simulink model "Inverter_pq_comp_sat_sim"  (R2023b)
settings: Solver=FixedStepDiscrete  StartTime=0.0  StopTime=2  RelTol=1e-3  EnableMultiTasking=on
InitFcn:
  | %% Definition of the parameters
  | 
  | Parameter_Definition
  | 
  | %% Damping
  | 
  | Rd = 3.9;
  | 
  | %% PRes Gains Calculation
  | 
  | % Definicao das grandezas
  | w_cl = 1j*2*pi*1200;  % Phase Crossing Frequency
  | no   = 1;           % Integral Resonant Constant
  | A    = 1;             % Carrier Amplitude
  | 
  | % Kp calculation
  | a0 = 1;
  | a1 = Rd*Cf;
  | b0 = 0;
  | b1 = Lf+Lg;
  | b2 = Rd*Lf*Cf+Rd*Lg*Cf;
  | b3 = Lf*Lg*Cf;
  | 
  | G_lcl = (a1*w_cl+a0)/(b3*w_cl^3+b2*w_cl^2+b1*w_cl+b0);
  | % G_lcl = 1/((Lf+Lg)*w_cl+Rf);
  | 
  | G_PWM = (1/A)*(1-w_cl*Ts/4)/(1+w_cl*Ts/4);
  | 
  | G_wc  = (Vdc/2)*(1/I_base)*G_lcl*G_PWM;
  | 
  | G_wc_abs = abs(G_wc);
  | 
  | Kp = 1/G_wc_abs;
  | 
  | % Discretized Controller Gains
  | ressonance_list = [1,5,7,11,13];
  | 
  | n_res = length(ressonance_list);
  | a = zeros(2,n_res);
  | b = zeros(2,n_res);
  | Ki_res = zeros(1,n_res);
  | 
  | % for i = 1:n_res
  | %   k = ressonance_list(i);
  | %   Ki_res(i) = (2.2*Kp)/(no*T_gr);
  | %   a(i) = (2*Ki_res(i)*Ts)/(4+((k*w_gr)^2)*Ts^2);
  | %   b(i) = (-8+2*((k*w_gr)^2)*Ts^2)/(4+((k*w_gr)^2)*Ts^2);
  | % end
  | 
  | % wc is the cutoff frequency/damping factor in rad/s
  | wc = 2;
  | 
  | for i = 1:n_res
  |   k = ressonance_list(i);
  |   wk = k * w_gr; % Resonant frequency for this harmonic
  | 
  |   Ki_res(i) = (2.2*Kp)/(0.8*no*T_gr);
  | 
  |   % 1. Calculate the common denominator
  |   den = 4 + 4*wc*Ts + (wk^2)*(Ts^2);
  | 
  |   % 2. Calculate the numerator terms (A coefficients for the input x)
  |   num_A0 = 2 * Ki_res(i) * wc * Ts;
  | 
  |   % 3. Calculate the denominator terms (B coefficients for the output y)
  |   num_B1 = -8 + 2*(wk^2)*(Ts^2);
  |   num_B2 = 4 - 4*wc*Ts + (wk^2)*(Ts^2);
  | 
  |   % 4. Normalize the coefficients
  |   a(1,i) = num_A0 / den;
  |   a(2,i) = -1*num_A0 / den;
  |   b(1,i) = num_B1 / den;
  |   b(2,i) = num_B2 / den;
  | end
values from neighbouring files (symbols this model uses):
  a1_sogi = single(2*(w0_sogi^2-c_sogi^2)/den0_sogi)    [Parameter_Definition.m]
  a2_sogi = single((c_sogi^2                 - k_sogi*w0_sogi*c_sogi                 + w0_sogi^2)/den0_sogi)    [Parameter_Definition.m]
  bD_sogi = single(k_sogi*w0_sogi*c_sogi/den0_sogi)    [Parameter_Definition.m]
  bQ_sogi = single(k_sogi*w0_sogi^2/den0_sogi)    [Parameter_Definition.m]
  Cdc = 1.5e-3    (= 0.0015)    [Parameter_Definition.m]
  Cf = 5e-6    (= 5e-06)    [Parameter_Definition.m]
  f_gr = 60    [Parameter_Definition.m]
  I_base = S_base/(sqrt(3)*V_gr)    [Parameter_Definition.m]
  Lf = 1e-3    (= 0.001)    [Parameter_Definition.m]
  Lg = 0.5e-3    (= 0.0005)    [Parameter_Definition.m]
  Rdc = 0.1/(2*pi*60*Cdc)    (= 0.176838825658)    [Parameter_Definition.m]
  Rf = 0.1*Xf    (= 0.0376991118431)    [Parameter_Definition.m]
  Rg = 0.1*Xg    (= 0.0188495559215)    [Parameter_Definition.m]
  S_base = S_rated    (= 1000)    [Parameter_Definition.m]
  Ts = 2*(4167)/100e6    (= 8.334e-05)    [Parameter_Definition.m]
  Tstep = Ts/1000    (= 8.334e-08)    [Parameter_Definition.m]
  V_base = sqrt(3)*V_gr    [Parameter_Definition.m]
  V_gr = 127    [Parameter_Definition.m]
  Vdc = 800    [Parameter_Definition.m]
  Vdc_base = Vdc    (= 800)    [Parameter_Definition.m]
  w_gr = 2*pi*f_gr    (= 376.991118431)    [Parameter_Definition.m]
undefined symbols (not defined in the file or in its folder): gH_LUT, gQ_LUT, gV_LUT, lH_vetor, lQ_vetor, lV_vetor
libraries: spsSeriesRLCBranchLib x22, spsIGBTDiodeLib x12, spsCurrentMeasurementLib x9, spsVoltageMeasurementLib x5, c2837xDlib x4, spsACVoltageSourceLib x3, spsGroundLib x3, spsDCVoltageSourceLib x2, spsTriangleGeneratorLib x1, simulink x1, eeRmsMeasurement x1, spsTHDLib x1
(part 1 of 3)
settings Model: SimulationMode=accelerator  ExtModeTrigDuration=8  Creator=AugustoMatheusdosSan  LastModifiedBy=engam
settings SolverCC: AutoInsertRateTranBlk=on
settings OptimizationCC: DefaultUnderspecifiedDataType=single  EnhancedBackFolding=on  PassReuseOutputArgsAs=Individual arguments  MaxStackSize=1024  OptimizeBlockOrder=speed  DifferentSizesBufferReuse=on  OptimizationCustomize=off  EfficientTunableParamExpr=on
settings DebuggingCC: ParameterPrecisionLossMsg=none  ParameterTunabilityLossMsg=error
settings HardwareCC: ProdBitPerChar=16  ProdBitPerInt=16  ProdBitPerPointer=32  ProdBitPerSizeT=32  ProdBitPerPtrDiffT=32  ProdLargestAtomicInteger=Integer  ProdLargestAtomicFloat=None  ProdWordSize=16  ProdLongLongMode=on  ProdHWDeviceType=Texas Instruments->C2000  HardwareBoardFeatureSet=SoCBlockset
settings ModelReferenceCC: ModelReferenceNumInstancesAllowed=Single
settings SFSimCC: MATLABDynamicMemAlloc=off
settings RTWCC: Description=Embedded Coder  SystemTargetFile=ert.tlc  HardwareBoard=TI Delfino F2837xD  TemplateMakefile=ert_default_tmf  Toolchain=Texas Instruments Code Composer Studio (C2000)  BuildConfiguration=Faster Runs  CodeProfilingSaveOptions=MetricsOnly
settings CodeAppCC: ForceParamTrailComments=on  IgnoreCustomStorageClasses=off  OperatorAnnotations=on  SimulinkDataObjDesc=on  SFDataObjDesc=on  InsertBlockDesc=on
settings ERTTargetCC: TargetLangStandard=C99 (ISO)  CodeReplacementLibrary=TI C28x  ExtModeTransport=4  ExtModeStaticAlloc=on  ExtModeAutomaticAllocSize=off  ExtModeStaticAllocSize=10000  ExtModeMexFile=ext_xcp  ExtModeIntrfLevel=Level2 - Open  EnableUserReplacementTypes=on

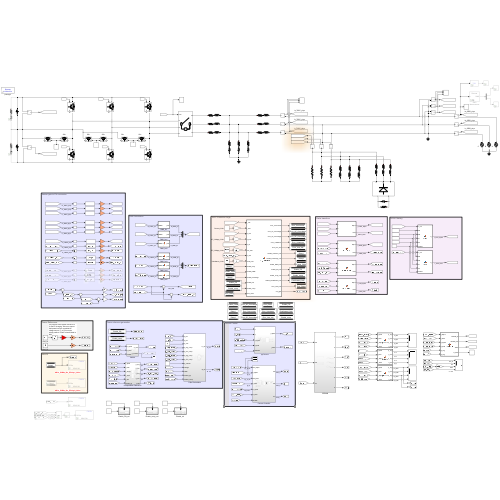
[thumbnail: Simulink's stored preview of the top-level diagram]
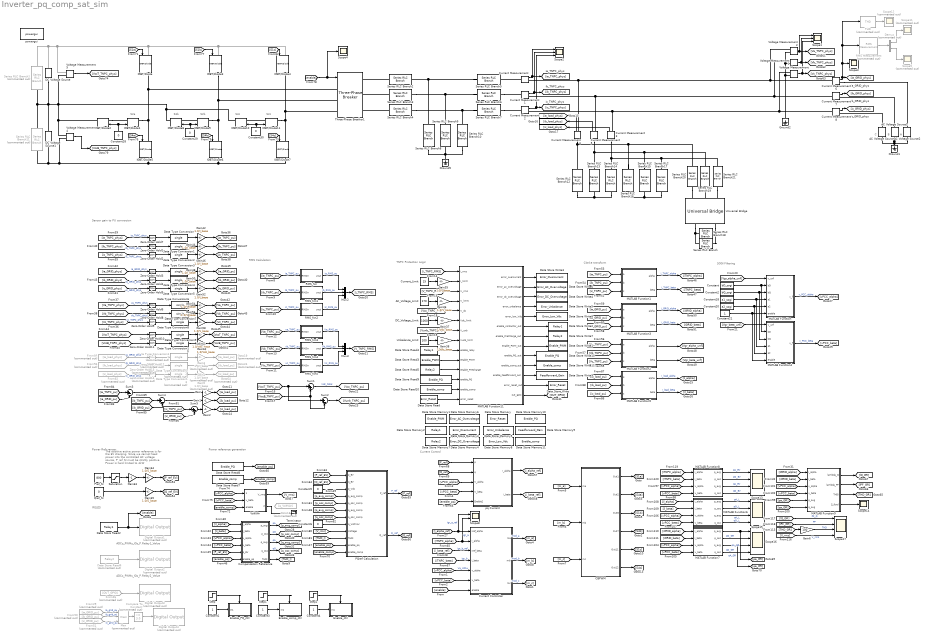
== system Inverter_pq_comp_sat_sim ==
  note: Power reference generation
  note: Current Control
  note: Power References
  note: The positive active power reference is for the EV charging. Since we cannot feed power into the controlled AC voltage source, P_ref_SI must be strictly positive. Power is hard limited to 4kW
  note: Sensor gain to PU conversion
  note: SOGI Filtering
  note: Clarke transform
  note: RELÉS
  note: ADCs_PWMs_IOs_P.Relay2_Value
  note: ADCs_PWMs_IOs_P.Relay1_Value
  note: RMS Calculation
  note: TNPC Protection Logic
  note: S3c
  note: S2b
  note: S2c
  note: S3b
  note: S2a
  note: C
  note: A
  note: B
  AC Voltage Source : spsACVoltageSourceLib/AC Voltage Source  Amplitude=V_gr*sqrt(2)  Phase=120  Frequency=f_gr  SampleTime=0  Measurements=None  BusType=swing  Pref=10e3  Qref=0  Qmin=-inf  Qmax=+inf
  AC Voltage Source1 : spsACVoltageSourceLib/AC Voltage Source  Amplitude=V_gr*sqrt(2)  Phase=-120  Frequency=f_gr  SampleTime=0  Measurements=None  BusType=swing  Pref=10e3  Qref=0  Qmin=-inf  Qmax=+inf
  AC Voltage Source2 : spsACVoltageSourceLib/AC Voltage Source  Amplitude=V_gr*sqrt(2)  Phase=0  Frequency=f_gr  SampleTime=0  Measurements=None  BusType=swing  Pref=10e3  Qref=0  Qmin=-inf  Qmax=+inf
  AC_Voltage_Limit : Constant  Value=170  OutDataTypeStr=single
  CBPWM : Subsystem
  Compare To Constant : simulink/Logic and Bit Operations/Compare To Constant  Commented=on  relop=<=  const=3.0  OutDataTypeStr=boolean
  Compensation Reference : Subsystem
  Constant : Constant  Value=bD_sogi
  Constant1 : Constant  OutDataTypeStr=single
  Constant18 : Constant  Value=a1_sogi
  Constant2 : Constant  Value=bQ_sogi
  Constant20 : Constant  Value=a2_sogi
  Constant21 : Constant
  Constant28 : Constant  Value=0
  Constant29 : Constant  Value=0
  Constant3 : Constant  OutDataTypeStr=single
  Constant30 : Constant  Value=0
  Constant4 : Constant  OutDataTypeStr=single
  Constant5 : Constant  Value=0  OutDataTypeStr=single
  Constant6 : Constant  Value=0  OutDataTypeStr=single
  Current Controller : Subsystem
  Current Measurement{,1..8} (9 alike) : spsCurrentMeasurementLib/Current Measurement  PhasorSimulation=off  OutputType=Complex  PSBequivalent=0
  Current_Limit : Constant  Value=15  OutDataTypeStr=single
  DC Voltage Source : spsDCVoltageSourceLib/DC Voltage Source  Amplitude=Vdc/2  Measurements=None
  DC Voltage Source1 : spsDCVoltageSourceLib/DC Voltage Source  Amplitude=Vdc/2  Measurements=None
  DC_Voltage_Limit : Constant  Value=1000  OutDataTypeStr=single
  Data Store Memory : DataStoreMemory  DataStoreName=Error_Reset  WriteAfterWriteMsg=warning  ShowAdditionalParam=off  OutDataTypeStr=single
  Data Store Memory1 : DataStoreMemory  DataStoreName=Enable_PWM  WriteAfterWriteMsg=warning  ShowAdditionalParam=off  OutDataTypeStr=single
  Data Store Memory10 : DataStoreMemory  DataStoreName=Enable_PQ  WriteAfterWriteMsg=warning  ShowAdditionalParam=off  OutDataTypeStr=single
  Data Store Memory11 : DataStoreMemory  DataStoreName=Enable_comp  WriteAfterWriteMsg=warning  ShowAdditionalParam=off  OutDataTypeStr=single
  Data Store Memory2 : DataStoreMemory  DataStoreName=Relay1  WriteAfterWriteMsg=warning  ShowAdditionalParam=off  OutDataTypeStr=single
  Data Store Memory3 : DataStoreMemory  DataStoreName=Error_Overcurrent  WriteAfterWriteMsg=warning  ShowAdditionalParam=off  OutDataTypeStr=single
  Data Store Memory4 : DataStoreMemory  DataStoreName=Error_DC_Overvoltage  WriteAfterWriteMsg=warning  ShowAdditionalParam=off  OutDataTypeStr=single
  Data Store Memory5 : DataStoreMemory  DataStoreName=Error_Unbalance  WriteAfterWriteMsg=warning  ShowAdditionalParam=off  OutDataTypeStr=single
  Data Store Memory6 : DataStoreMemory  DataStoreName=Error_AC_Overvoltage  WriteAfterWriteMsg=warning  ShowAdditionalParam=off  OutDataTypeStr=single
  Data Store Memory7 : DataStoreMemory  DataStoreName=Relay2  WriteAfterWriteMsg=warning  ShowAdditionalParam=off  OutDataTypeStr=single
  Data Store Memory8 : DataStoreMemory  DataStoreName=Error_Low_Vdc  WriteAfterWriteMsg=warning  ShowAdditionalParam=off  OutDataTypeStr=single
  Data Store Memory9 : DataStoreMemory  DataStoreName=Feedforward_Gain  WriteAfterWriteMsg=warning  ShowAdditionalParam=off  OutDataTypeStr=single
  Data Store Read : DataStoreRead  DataStoreName=Error_Reset  SampleTime=Ts  IndexOptions=Index vector (dialog)  Indices=1  OutputSizes=1
  Data Store Read10 : DataStoreRead  DataStoreName=Enable_comp  SampleTime=Ts  IndexOptions=Index vector (dialog)  Indices=1  OutputSizes=1
  Data Store Read2 : DataStoreRead  DataStoreName=Relay1  SampleTime=Ts  IndexOptions=Index vector (dialog)  Indices=1  OutputSizes=1
  Data Store Read3 : DataStoreRead  DataStoreName=Enable_PWM  SampleTime=Ts  IndexOptions=Index vector (dialog)  Indices=1  OutputSizes=1
  Data Store Read4 : DataStoreRead  DataStoreName=Relay1  SampleTime=Ts  IndexOptions=Index vector (dialog)  Indices=1  OutputSizes=1
  Data Store Read5 : DataStoreRead  DataStoreName=Relay2  SampleTime=Ts  IndexOptions=Index vector (dialog)  Indices=1  OutputSizes=1
  Data Store Read6 : DataStoreRead  Commented=on  DataStoreName=Relay2  IndexOptions=Index vector (dialog)  Indices=1  OutputSizes=1
  Data Store Read7 : DataStoreRead  DataStoreName=Enable_comp  SampleTime=Ts  IndexOptions=Index vector (dialog)  Indices=1  OutputSizes=1
  Data Store Read8 : DataStoreRead  DataStoreName=Enable_PQ  SampleTime=Ts  IndexOptions=Index vector (dialog)  Indices=1  OutputSizes=1
  Data Store Read9 : DataStoreRead  DataStoreName=Enable_PQ  SampleTime=Ts  IndexOptions=Index vector (dialog)  Indices=1  OutputSizes=1
  Data Store Write : DataStoreWrite  DataStoreName=Error_Reset  SampleTime=Ts  IndexOptions=Index vector (dialog)  Indices=1  OutputSizes=1
  Data Store Write1 : DataStoreWrite  DataStoreName=Enable_PWM  SampleTime=Ts  IndexOptions=Index vector (dialog)  Indices=1  OutputSizes=1
  Data Store Write10 : DataStoreWrite  DataStoreName=Enable_PQ  SampleTime=Ts  IndexOptions=Index vector (dialog)  Indices=1  OutputSizes=1
  Data Store Write11 : DataStoreWrite  DataStoreName=Enable_comp  SampleTime=Ts  IndexOptions=Index vector (dialog)  Indices=1  OutputSizes=1
  Data Store Write2 : DataStoreWrite  DataStoreName=Relay1  SampleTime=Ts  IndexOptions=Index vector (dialog)  Indices=1  OutputSizes=1
  Data Store Write3 : DataStoreWrite  DataStoreName=Error_Overcurrent  SampleTime=Ts  IndexOptions=Index vector (dialog)  Indices=1  OutputSizes=1
  Data Store Write4 : DataStoreWrite  DataStoreName=Error_DC_Overvoltage  SampleTime=Ts  IndexOptions=Index vector (dialog)  Indices=1  OutputSizes=1
  Data Store Write5 : DataStoreWrite  DataStoreName=Error_Unbalance  SampleTime=Ts  IndexOptions=Index vector (dialog)  Indices=1  OutputSizes=1
  Data Store Write6 : DataStoreWrite  DataStoreName=Error_AC_Overvoltage  SampleTime=Ts  IndexOptions=Index vector (dialog)  Indices=1  OutputSizes=1
  Data Store Write7 : DataStoreWrite  DataStoreName=Relay2  SampleTime=Ts  IndexOptions=Index vector (dialog)  Indices=1  OutputSizes=1
  Data Store Write8 : DataStoreWrite  DataStoreName=Error_Low_Vdc  SampleTime=Ts  IndexOptions=Index vector (dialog)  Indices=1  OutputSizes=1
  Data Store Write9 : DataStoreWrite  DataStoreName=Feedforward_Gain  SampleTime=Ts  IndexOptions=Index vector (dialog)  Indices=1  OutputSizes=1
  Data Type Conversion{,1..10} (11 alike) : DataTypeConversion  OutDataTypeStr=single  SaturateOnIntegerOverflow=off  RndMeth=Floor
  Data Type Conversion11 : DataTypeConversion  Commented=on  OutDataTypeStr=single  SaturateOnIntegerOverflow=off  RndMeth=Floor
  Data Type Conversion12 : DataTypeConversion  Commented=on  OutDataTypeStr=single  SaturateOnIntegerOverflow=off  RndMeth=Floor
  Data Type Conversion13 : DataTypeConversion  Commented=on  OutDataTypeStr=single  SaturateOnIntegerOverflow=off  RndMeth=Floor
  Demux : Demux  Commented=on  Outputs=2
  Digital Output1 : c2837xDlib/Digital Output  Commented=on  GPIO_Number=GPIO32~GPIO39  GPIO_Bit0=off  GPIO_BIT0_Toggle=off  GPIO_Bit1=off  GPIO_BIT1_Toggle=off  GPIO_Bit2=off  GPIO_BIT2_Toggle=off  GPIO_Bit3=on  GPIO_BIT3_Toggle=off  GPIO_Bit4=off  GPIO_BIT4_Toggle=off  GPIO_Bit5=off  GPIO_BIT5_Toggle=off  GPIO_Bit6=off  GPIO_BIT6_Toggle=off  GPIO_Bit7=off  GPIO_BIT7_Toggle=off
  Digital Output2 : c2837xDlib/Digital Output  Commented=on  GPIO_Number=GPIO32~GPIO39  GPIO_Bit0=off  GPIO_BIT0_Toggle=off  GPIO_Bit1=off  GPIO_BIT1_Toggle=off  GPIO_Bit2=off  GPIO_BIT2_Toggle=off  GPIO_Bit3=off  GPIO_BIT3_Toggle=off  GPIO_Bit4=off  GPIO_BIT4_Toggle=off  GPIO_Bit5=on  GPIO_BIT5_Toggle=off  GPIO_Bit6=off  GPIO_BIT6_Toggle=off  GPIO_Bit7=off  GPIO_BIT7_Toggle=off
  Digital Output3 : c2837xDlib/Digital Output  Commented=on  GPIO_Number=GPIO64~GPIO71  GPIO_Bit0=off  GPIO_BIT0_Toggle=off  GPIO_Bit1=off  GPIO_BIT1_Toggle=off  GPIO_Bit2=off  GPIO_BIT2_Toggle=off  GPIO_Bit3=on  GPIO_BIT3_Toggle=off  GPIO_Bit4=off  GPIO_BIT4_Toggle=off  GPIO_Bit5=off  GPIO_BIT5_Toggle=off  GPIO_Bit6=off  GPIO_BIT6_Toggle=off  GPIO_Bit7=off  GPIO_BIT7_Toggle=off
  Digital Output4 : c2837xDlib/Digital Output  Commented=on  GPIO_Number=GPIO64~GPIO71  GPIO_Bit0=off  GPIO_BIT0_Toggle=off  GPIO_Bit1=off  GPIO_BIT1_Toggle=off  GPIO_Bit2=off  GPIO_BIT2_Toggle=off  GPIO_Bit3=off  GPIO_BIT3_Toggle=off  GPIO_Bit4=on  GPIO_BIT4_Toggle=off  GPIO_Bit5=off  GPIO_BIT5_Toggle=off  GPIO_Bit6=off  GPIO_BIT6_Toggle=off  GPIO_Bit7=off  GPIO_BIT7_Toggle=off
  Enable_PQ_ctrl : Subsystem  TreatAsAtomicUnit=on
  Enable_comp_ctrl : Subsystem  TreatAsAtomicUnit=on
  Enable_ctrl : Subsystem  TreatAsAtomicUnit=on
  From26 : From  Commented=on  GotoTag=OUT_GPIO
  From29 : From  Commented=on  GotoTag=ia_GRID_pu
  From50 : From  Commented=on  GotoTag=ib_GRID_pu
  From51 : From  Commented=on  GotoTag=ic_GRID_pu
  From92 : From  Commented=on  GotoTag=ic_load_phys
  From93 : From  Commented=on  GotoTag=ia_load_phys
  From94 : From  Commented=on  GotoTag=ib_load_phys
  Gain{,1..2,63} (4 alike) : Gain  Gain=-1
  Gain3 : Gain  Commented=on  Gain=1.0/I_base
  Gain{35,42,44,46,48,50,52} (7 alike) : Gain  Gain=1.0/I_base
  Gain{36,54,56,58} (4 alike) : Gain  Gain=1.0/V_base
  Gain37 : Gain  Gain=1/Vdc_base
  Gain38 : Gain  Gain=1/Vdc_base
  Gain4 : Gain  Commented=on  Gain=1.0/I_base
  Gain5 : Gain  Commented=on  Gain=1.0/I_base
  Gain6 : Gain  Gain=100
  Gain61 : Gain  Gain=1.0/Vdc_base
  Gain62 : Gain  Gain=1.0/Vdc_base
  Gain64 : Gain  Gain=1.0/S_base
  Gain65 : Gain  Gain=1.0/S_base
  Goto18 : Goto  Commented=on  GotoTag=q_VoltVAr
  Goto19 : Goto  Commented=on  GotoTag=ia_load_pu
  Goto24 : Goto  Commented=on  GotoTag=ib_load_pu
  Goto64 : Goto  Commented=on  GotoTag=ic_load_pu
  Ground1 : spsGroundLib/Ground  LConnTagsString=a
  Ground2 : spsGroundLib/Ground  LConnTagsString=a
  Ground5 : spsGroundLib/Ground  LConnTagsString=a
  IGBT/Diode{,1..11} (12 alike) : spsIGBTDiodeLib/IGBT//Diode  Ron=Rfet  Rs=1e5  Cs=inf  Measurements=on
  MATLAB Function : MATLAB Function  TreatAsAtomicUnit=on
  MATLAB Function1 : MATLAB Function  TreatAsAtomicUnit=on
  MATLAB Function11 : MATLAB Function  TreatAsAtomicUnit=on
  MATLAB Function2 : MATLAB Function  TreatAsAtomicUnit=on
  MATLAB Function3 : MATLAB Function  TreatAsAtomicUnit=on
  MATLAB Function4 : MATLAB Function  TreatAsAtomicUnit=on
  MATLAB Function5 : MATLAB Function  TreatAsAtomicUnit=on
  MATLAB Function6 : MATLAB Function  TreatAsAtomicUnit=on
  MATLAB Function7 : MATLAB Function  TreatAsAtomicUnit=on
  MATLAB Function8 : MATLAB Function  TreatAsAtomicUnit=on
  MATLAB Function9 : MATLAB Function  TreatAsAtomicUnit=on
  Max : MinMax  Commented=on  Function=max  Inputs=3
  Mux2 : Mux  Inputs=3
  Mux3 : Mux  Inputs=3
  PQref Calculation : Subsystem
  Pref_SI : Constant  Value=800  OutDataTypeStr=single
  Qref_SI : Constant  Value=0  OutDataTypeStr=single
  RMS Measurement : eeRmsMeasurement/RMS Measurement  Commented=on  LabelModeActiveChoice=Harmonic  F=60  SpecifyHarmonics=on  K=[1:40]  Ts=Ts
      settings: LibrarySourceBlock=|
      | ee_sl_lib/Measurements/RMS
      | Measurement
  RMS_fcn : MATLAB Function  TreatAsAtomicUnit=on
  RMS_fcn1 : MATLAB Function  TreatAsAtomicUnit=on
  RMS_fcn2 : MATLAB Function  TreatAsAtomicUnit=on
  RMS_fcn3 : MATLAB Function  TreatAsAtomicUnit=on
  RMS_fcn4 : MATLAB Function  TreatAsAtomicUnit=on
  RMS_fcn5 : MATLAB Function  TreatAsAtomicUnit=on
  Saturation : Saturate  UpperLimit=4000  LowerLimit=0
  Scope1 : Scope  NumInputPorts=3
  Scope11 : Scope  Commented=on
  Scope12 : Scope  Commented=on
  Scope{13,15..17} (4 alike) : Scope  NumInputPorts=4
  Scope14 : Scope
  Scope2 : Scope  NumInputPorts=3
  Scope3 : Scope
  Scope4 : Scope
  Scope5 : Scope  Commented=on
  Scope8 : Scope  NumInputPorts=2
  Series RLC Branch : spsSeriesRLCBranchLib/Series RLC Branch  LConnTagsString=__new0  RConnTagsString=__new0  BranchType=R  Resistance=400  Inductance=1e-3  SetiL0=off  InitialCurrent=0  Capacitance=1e-6  Setx0=off  InitialVoltage=0  Measurements=None
  Series RLC Branch1 : spsSeriesRLCBranchLib/Series RLC Branch  Commented=on  LConnTagsString=__new0  RConnTagsString=__new0  BranchType=RC  Resistance=Rdc*0.1  Inductance=Cdc  SetiL0=off  InitialCurrent=0  Capacitance=Cdc  Setx0=on  InitialVoltage=Vdc/2  Measurements=None
  Series RLC Branch10 : spsSeriesRLCBranchLib/Series RLC Branch  LConnTagsString=__new0  RConnTagsString=__new0  BranchType=RC  Resistance=Rd  Inductance=5e-3  SetiL0=off  InitialCurrent=0  Capacitance=Cf  Setx0=off  InitialVoltage=0  Measurements=None
  Series RLC Branch11 : spsSeriesRLCBranchLib/Series RLC Branch  Commented=on  LConnTagsString=__new0  RConnTagsString=__new0  BranchType=RC  Resistance=Rdc*0.1  Inductance=Cdc  SetiL0=off  InitialCurrent=0  Capacitance=Cdc  Setx0=on  InitialVoltage=Vdc/2  Measurements=None
  Series RLC Branch12 : spsSeriesRLCBranchLib/Series RLC Branch  LConnTagsString=__new0  RConnTagsString=__new0  BranchType=R  Resistance=80*160/240  Inductance=5e-3  SetiL0=off  InitialCurrent=0  Capacitance=inf  Setx0=off  InitialVoltage=0  Measurements=None
  Series RLC Branch13 : spsSeriesRLCBranchLib/Series RLC Branch  LConnTagsString=__new0  RConnTagsString=__new0  BranchType=R  Resistance=80*160/240  Inductance=5e-3  SetiL0=off  InitialCurrent=0  Capacitance=inf  Setx0=off  InitialVoltage=0  Measurements=None
  Series RLC Branch14 : spsSeriesRLCBranchLib/Series RLC Branch  LConnTagsString=__new0  RConnTagsString=__new0  BranchType=R  Resistance=80*160/240  Inductance=5e-3  SetiL0=off  InitialCurrent=0  Capacitance=inf  Setx0=off  InitialVoltage=0  Measurements=None
  Series RLC Branch15 : spsSeriesRLCBranchLib/Series RLC Branch  LConnTagsString=__new0  RConnTagsString=__new0  BranchType=RL  Resistance=5.47  Inductance=188.7e-3  SetiL0=off  InitialCurrent=0  Capacitance=inf  Setx0=off  InitialVoltage=0  Measurements=None
  Series RLC Branch16 : spsSeriesRLCBranchLib/Series RLC Branch  LConnTagsString=__new0  RConnTagsString=__new0  BranchType=RL  Resistance=5.47  Inductance=188.7e-3  SetiL0=off  InitialCurrent=0  Capacitance=inf  Setx0=off  InitialVoltage=0  Measurements=None
  Series RLC Branch17 : spsSeriesRLCBranchLib/Series RLC Branch  LConnTagsString=__new0  RConnTagsString=__new0  BranchType=RL  Resistance=5.47  Inductance=188.7e-3  SetiL0=off  InitialCurrent=0  Capacitance=inf  Setx0=off  InitialVoltage=0  Measurements=None
  Series RLC Branch18 : spsSeriesRLCBranchLib/Series RLC Branch  LConnTagsString=__new0  RConnTagsString=__new0  BranchType=C  Resistance=(54/pi^2)*(127^2/1e3)  Inductance=1e-3  SetiL0=off  InitialCurrent=0  Capacitance=5e-3  Setx0=off  InitialVoltage=0  Measurements=None
  Series RLC Branch19 : spsSeriesRLCBranchLib/Series RLC Branch  LConnTagsString=__new0  RConnTagsString=__new0  BranchType=RL  Resistance=0.1*2*pi*60*1e-3  Inductance=1e-3  SetiL0=off  InitialCurrent=0  Capacitance=5e-6  Setx0=off  InitialVoltage=0  Measurements=None
  Series RLC Branch2 : spsSeriesRLCBranchLib/Series RLC Branch  LConnTagsString=__new0  RConnTagsString=__new0  BranchType=RL  Resistance=Rf  Inductance=Lf  SetiL0=off  InitialCurrent=0  Capacitance=1e-6  Setx0=off  InitialVoltage=0  Measurements=None
  Series RLC Branch20 : spsSeriesRLCBranchLib/Series RLC Branch  LConnTagsString=__new0  RConnTagsString=__new0  BranchType=RL  Resistance=0.1*2*pi*60*1e-3  Inductance=1e-3  SetiL0=off  InitialCurrent=0  Capacitance=5e-6  Setx0=off  InitialVoltage=0  Measurements=None
  Series RLC Branch21 : spsSeriesRLCBranchLib/Series RLC Branch  LConnTagsString=__new0  RConnTagsString=__new0  BranchType=RL  Resistance=0.1*2*pi*60*1e-3  Inductance=1e-3  SetiL0=off  InitialCurrent=0  Capacitance=5e-6  Setx0=off  InitialVoltage=0  Measurements=None
  Series RLC Branch3 : spsSeriesRLCBranchLib/Series RLC Branch  LConnTagsString=__new0  RConnTagsString=__new0  BranchType=RL  Resistance=Rf  Inductance=Lf  SetiL0=off  InitialCurrent=0  Capacitance=1e-6  Setx0=off  InitialVoltage=0  Measurements=None
  Series RLC Branch4 : spsSeriesRLCBranchLib/Series RLC Branch  LConnTagsString=__new0  RConnTagsString=__new0  BranchType=RL  Resistance=Rf  Inductance=Lf  SetiL0=off  InitialCurrent=0  Capacitance=1e-6  Setx0=off  InitialVoltage=0  Measurements=None
  Series RLC Branch5 : spsSeriesRLCBranchLib/Series RLC Branch  LConnTagsString=__new0  RConnTagsString=__new0  BranchType=RL  Resistance=Rg  Inductance=Lg  SetiL0=off  InitialCurrent=0  Capacitance=1e-6  Setx0=off  InitialVoltage=0  Measurements=None
  Series RLC Branch6 : spsSeriesRLCBranchLib/Series RLC Branch  LConnTagsString=__new0  RConnTagsString=__new0  BranchType=RL  Resistance=Rg  Inductance=Lg  SetiL0=off  InitialCurrent=0  Capacitance=1e-6  Setx0=off  InitialVoltage=0  Measurements=None
  Series RLC Branch7 : spsSeriesRLCBranchLib/Series RLC Branch  LConnTagsString=__new0  RConnTagsString=__new0  BranchType=RL  Resistance=Rg  Inductance=Lg  SetiL0=off  InitialCurrent=0  Capacitance=1e-6  Setx0=off  InitialVoltage=0  Measurements=None
  Series RLC Branch8 : spsSeriesRLCBranchLib/Series RLC Branch  LConnTagsString=__new0  RConnTagsString=__new0  BranchType=RC  Resistance=Rd  Inductance=5e-3  SetiL0=off  InitialCurrent=0  Capacitance=Cf  Setx0=off  InitialVoltage=0  Measurements=None
  Series RLC Branch9 : spsSeriesRLCBranchLib/Series RLC Branch  LConnTagsString=__new0  RConnTagsString=__new0  BranchType=RC  Resistance=Rd  Inductance=5e-3  SetiL0=off  InitialCurrent=0  Capacitance=Cf  Setx0=off  InitialVoltage=0  Measurements=None
  Step : Step  OutDataTypeStr=single  SampleTime=Ts
  Step1 : Step  Time=1.5  OutDataTypeStr=single  SampleTime=Ts
  Step2 : Step  Time=0.5  OutDataTypeStr=single  SampleTime=Ts
  Sum1 : Sum  Inputs=|++
  Sum{2..5} (4 alike) : Sum  Inputs=|+-
  THD : spsTHDLib/THD  Commented=on  Freq=60  Ts=Tstep
  Terminator : Terminator
  Three-Phase Breaker1 : spsThreePhaseBreakerLib/Three-Phase Breaker  InitialState=open  SwitchA=on  SwitchB=on  SwitchC=on  SwitchTimes="[1/60  5/60]"  External=on  BreakerResistance=0.001  SnubberResistance=1e6  SnubberCapacitance=inf  Measurements=None
  Unbalance_Limit : Constant  Value=100  OutDataTypeStr=single
  Universal Bridge : spsUniversalBridgeLib/Universal Bridge  Arms=3  SnubberResistance=1e5  SnubberCapacitance=inf  Device=Diodes  Ron=1e-3  Lon=0  ForwardVoltages="[  0  0  ]"  ForwardVoltage=0  GTOparameters=[ 10e-6 , 20e-6 ]  IGBTparameters=[ 1e-6 , 2e-6 ]  Measurements=None  Measurements_2=None  converterType=Rectifier
  VoltVAr : Subsystem
  Voltage Measurement{,1..2,4..5} (5 alike) : spsVoltageMeasurementLib/Voltage Measurement  PhasorSimulation=off  OutputType=Complex  PSBequivalent=0
  Zero-Order Hold{1..11} (11 alike) : ZeroOrderHold  SampleTime=Ts
  Zero-Order Hold12 : ZeroOrderHold  Commented=on  SampleTime=Ts
  Zero-Order Hold13 : ZeroOrderHold  Commented=on  SampleTime=Ts
  Zero-Order Hold14 : ZeroOrderHold  Commented=on  SampleTime=Ts
  powergui : sps_lib/powergui  Priority=1  SimulationMode=Discrete  SampleTime=Tstep  frequency=60  Iterations=50  frequencyindice=60  Pbase=100e6  ErrMax=1e-4  UnitsV=kV  UnitsW=MW  buscounter=0  FunctionMessages=off  echomessages=off  EnableUseOfTLC=off  CurrentSourceSwitches=off  DisableSnubberDevices=off  DisableRonSwitches=off  DisableVfSwitches=off  DisplayEquations=off  AutomaticDiscreteSolvers=off  SolverType=Tustin/Backward Euler (TBE)  Interpol=off  ExternalGateDelay=off  methode=off  Ts=100  x0status=blocks  SPID=on  SwTol=0  HookPort=off  NonlinearTolerance=1e-4  nMaxIteration=100  ContinueOnMaxIteration=off  RestoreLinks=warning  ResistiveCurrentMeasurement=off  Frange=[0:2:500]  Ylog=off  Xlog=on  ShowGrid=off  save=off  variable=ZData  structure=0  ZoomFFT=off  StartTime=0.0  cycles=1  DisplayStyle=1  fundamental=60  FreqAxis=off  MaxFrequency=1000  frequencyindicesteady=1  RmsSteady=1  display=off
  pq Current : Subsystem
  wires:
  [iTNPC_alpha] -> Scope8/2, Current Controller/2(i_alpha)  "igr_a"
  [i_alpha_ref] -> Scope8/1, Current Controller/1(iref_alpha)  "igr_a_ref"
  [iTNPC_beta] -> Current Controller/4(i_beta)  "igr_b"
  [i_beta_ref] -> Current Controller/3(iref_beta)  "igr_b_ref"
  Current Controller/3(mc) -> [m_c]  "mod_c"
  Data Store Read6/1 -> Digital Output2/1
  Current Controller/2(mb) -> [m_b]  "mod_b"
  [enable] -> Current Controller/7(enable)
  Current Controller/1(ma) -> [m_a]  "mod_a"
  Data Store Read/1 -> MATLAB Function11/14(error_reset)
  [ib_TNPC_pu] -> RMS_fcn1/1(RMSin)  "ib_TNPC_pu"
  Data Store Read5/1 -> MATLAB Function11/11(enable_PreCharge)
  AC_Voltage_Limit/1 -> Gain36/1
  [ia_TNPC_pu] -> RMS_fcn/1(RMSin)  "ia_TNPC_pu"
  [VccB_TNPC_pu] -> Sum1/2, Sum2/2
  Data Store Read3/1 -> MATLAB Function11/10(enable_PWM)
  DC_Voltage_Limit/1 -> Gain37/1
  Gain35/1 -> MATLAB Function11/2(I_limit)
  Mux2/1 -> [i_TNPC_RMS]
  Unbalance_Limit/1 -> Gain38/1
  MATLAB Function11/8(enable_PWM_out) -> Data Store Write1/1
  [ic_TNPC_pu] -> RMS_fcn2/1(RMSin)  "ic_TNPC_pu"
  [Vcc_TNPC_pu] -> MATLAB Function11/5(V_dc)
  Gain36/1 -> MATLAB Function11/4(V_limit)
  MATLAB Function11/1(error_overcurrent) -> Data Store Write3/1
  [V_TNPC_RMS] -> MATLAB Function11/3(V_rms)
  Sum2/1 -> [Vunb_TNPC_pu]
  Gain38/1 -> MATLAB Function11/8(Vunb_limit)
  Gain37/1 -> MATLAB Function11/6(Vdc_limit)
  Data Store Read4/1 -> MATLAB Function11/9(enable_relay)
  Current_Limit/1 -> Gain35/1
  MATLAB Function11/7(enable_PreCharge_out) -> Data Store Write7/1
  MATLAB Function11/6(enable_contactor_out) -> Data Store Write2/1
  [i_TNPC_RMS] -> MATLAB Function11/1(i_rms)
  Sum1/1 -> [Vcc_TNPC_pu]  "Vdc_total"
  [Vunb_TNPC_pu] -> MATLAB Function11/7(V_unb)
  [VccT_TNPC_pu] -> Sum1/1, Sum2/1
  MATLAB Function11/12(error_reset_out) -> Data Store Write/1
  MATLAB Function11/3(error_dc_overvoltage) -> Data Store Write4/1
  MATLAB Function11/4(error_unbalance) -> Data Store Write5/1
  RMS_fcn/1(yout) -> Mux2/1  "ia_RMS_pu"
  RMS_fcn1/1(yout) -> Mux2/2  "ib_RMS_pu"
  RMS_fcn2/1(yout) -> Mux2/3  "ic_RMS_pu"
  [Va_TNPC_pu] -> RMS_fcn3/1(RMSin)  "va_TNPC_pu"
  [Vc_TNPC_pu] -> RMS_fcn5/1(RMSin)  "vc_TNPC_pu"
  [Vb_TNPC_pu] -> RMS_fcn4/1(RMSin)  "vb_TNPC_pu"
  RMS_fcn4/1(yout) -> Mux3/2  "Vb_RMS_pu"
  RMS_fcn3/1(yout) -> Mux3/1  "Va_RMS_pu"
  RMS_fcn5/1(yout) -> Mux3/3  "Vc_RMS_pu"
  Mux3/1 -> [V_TNPC_RMS]
  MATLAB Function11/2(error_ac_overvoltage) -> Data Store Write6/1
  MATLAB Function11/5(error_low_Vdc) -> Data Store Write8/1
  MATLAB Function11/13(out_gpio) -> [OUT_GPIO]
  From26/1 -> Digital Output3/1
  [vPCC_alpha] -> Current Controller/5(v_alpha)  "Va_inPLL"
  [vPCC_beta] -> Current Controller/6(v_beta)
  Data Store Read2/1 -> [enable], Digital Output1/1
  Compare To Constant/1 -> Digital Output4/1
  MATLAB Function11/11(enable_Feedforward_out) -> Data Store Write9/1
  From29/1 -> Max/1  "ia_grid_pu"
  Max/1 -> Compare To Constant/1
  From50/1 -> Max/2  "ib_grid_pu"
  From51/1 -> Max/3  "ic_grid_pu"
  [ia_TNPC_pu] -> MATLAB Function1/1(a)
  [ib_TNPC_pu] -> MATLAB Function1/2(b)
  [ic_TNPC_pu] -> MATLAB Function1/3(c)
  [Va_TNPC_pu] -> MATLAB Function2/1(a)
  [Vb_TNPC_pu] -> MATLAB Function2/2(b)
  [Vc_TNPC_pu] -> MATLAB Function2/3(c)
  MATLAB Function1/2(beta) -> [iTNPC_beta]  "i_TNPC_beta"
  MATLAB Function1/1(alpha) -> [iTNPC_alpha]  "i_TNPC_alpha"
  MATLAB Function2/1(alpha) -> [Vgr_alpha_unf]
  MATLAB Function2/2(beta) -> [Vgr_beta_unf]
  [ib_GRID_pu] -> MATLAB Function3/2(b)
  [ia_GRID_pu] -> MATLAB Function3/1(a)
  MATLAB Function3/2(beta) -> [iGRID_beta]  "i_GRID_beta"
  MATLAB Function3/1(alpha) -> [iGRID_alpha]  "i_GRID_alpha"
  [ic_GRID_pu] -> MATLAB Function3/3(c)
  [Vgr_beta_unf] -> MATLAB Function4/1(v_unf)
  [Vgr_alpha_unf] -> MATLAB Function/1(v_unf)
  MATLAB Function4/1(v_f) -> [vPCC_beta]  "v_PCC_beta"
  MATLAB Function/1(v_f) -> [vPCC_alpha]  "v_PCC_alpha"
  Constant/1 -> MATLAB Function4/2(bD), MATLAB Function/2(bD)
  Constant2/1 -> MATLAB Function4/3(bQ), MATLAB Function/3(bQ)
  Constant18/1 -> MATLAB Function4/4(a1), MATLAB Function/4(a1)
  Constant20/1 -> MATLAB Function4/5(a2), MATLAB Function/5(a2)
  Constant21/1 -> MATLAB Function4/6(enable), MATLAB Function/6(enable)
  [enable_pq] -> Compensation Reference/6(enable_pq)
  Compensation Reference/3(q_avg) -> [q_avg_comp]  "qA"
  [vPCC_beta] -> Compensation Reference/4(v_beta)
  Compensation Reference/4(q_osc) -> [q_osc_comp]  "qO"
  Compensation Reference/1(p_avg) -> [p_avg_comp]  "pA"
  [il_beta] -> Compensation Reference/2(i_beta)
  [il_alpha] -> Compensation Reference/1(i_alpha)
  [P_ref_EV] -> Compensation Reference/5(p_EV)
  Compensation Reference/5(THDi) -> [THD_i]
  [vPCC_alpha] -> Compensation Reference/3(v_alpha)
  Compensation Reference/2(p_osc) -> [p_osc_comp]  "pO"
  [ia_TNPC_phys] -> Zero-Order Hold7/1  "ia_TNPC_phys"
  [ib_TNPC_phys] -> Zero-Order Hold1/1  "ib_TNPC_phys"
  [ic_TNPC_phys] -> Zero-Order Hold2/1  "ic_TNPC_phys"
  Gain42/1 -> [ia_TNPC_pu]
  Gain44/1 -> [ib_TNPC_pu]
  Gain46/1 -> [ic_TNPC_pu]
  Gain52/1 -> [ic_GRID_pu]
  Gain50/1 -> [ib_GRID_pu]
  [ic_GRID_phys] -> Zero-Order Hold5/1  "ic_GRID_phys"
  [ib_GRID_phys] -> Zero-Order Hold4/1  "ib_GRID_phys"
  [ia_GRID_phys] -> Zero-Order Hold3/1  "ia_GRID_phys"
  Gain48/1 -> [ia_GRID_pu]
  [Va_TNPC_phys] -> Zero-Order Hold6/1  "va_TNPC_phys"
  [Vb_TNPC_phys] -> Zero-Order Hold8/1  "vb_TNPC_phys"
  [Vc_TNPC_phys] -> Zero-Order Hold9/1  "vc_TNPC_phys"
  Gain54/1 -> [Va_TNPC_pu]
  Gain56/1 -> [Vb_TNPC_pu]
  Gain58/1 -> [Vc_TNPC_pu]
  [VccT_TNPC_phys] -> Zero-Order Hold10/1
  Gain61/1 -> [VccT_TNPC_pu]
  [VccB_TNPC_phys] -> Zero-Order Hold11/1
  Gain62/1 -> [VccB_TNPC_pu]
  Pref_SI/1 -> Saturation/1
  Saturation/1 -> Gain63/1
  Gain63/1 -> Gain64/1
  Qref_SI/1 -> Gain65/1
  Gain64/1 -> [P_ref_EV]
  Gain65/1 -> [Q_ref_EV]
  [P_ref_EV] -> PQref Calculation/1(p_EV)
  PQref Calculation/2(Q_ref) -> [Q_ref]  "Q_ref"
  [Q_ref_EV] -> PQref Calculation/2(q_EV)
  [p_avg_comp] -> PQref Calculation/4(p_avg_comp)
  PQref Calculation/1(P_ref) -> [P_ref]  "P_ref"
  [enable_pq] -> PQref Calculation/11(enable_pq)
  [P_ref] -> pq Current/1(p)
  [enable_pq] -> pq Current/5(Enable2)
  [Q_ref] -> pq Current/2(q)
  [vPCC_alpha] -> pq Current/3(V_alpha)
  pq Current/2(i_beta) -> [i_beta_ref]
  [vPCC_beta] -> pq Current/4(V_beta)
  pq Current/1(i_alpha) -> [i_alpha_ref]
  [enable_comp] -> PQref Calculation/12(enable_comp)
  Data Store Read7/1 -> [enable_comp]
  Data Store Read8/1 -> [enable_pq]
  Data Store Read10/1 -> MATLAB Function11/13(enable_comp)
  Data Store Read9/1 -> MATLAB Function11/12(enable_PQ)
  MATLAB Function11/9(enable_PQ_out) -> Data Store Write10/1
  MATLAB Function11/10(enable_comp_out) -> Data Store Write11/1
  Current Measurement1/1 -> Scope2/2, [ib_TNPC_phys]
  [enable] -> Scope4/1, Three-Phase Breaker1/1
  Constant28/1 -> IGBT/Diode2/1, IGBT/Diode1/1
  Voltage Measurement/1 -> [Vc_TNPC_phys], Scope1/3
  Constant29/1 -> IGBT/Diode8/1, IGBT/Diode9/1
  Current Measurement2/1 -> Scope2/3, [ic_TNPC_phys]
  Constant30/1 -> IGBT/Diode10/1, IGBT/Diode11/1
  Current Measurement6/1 -> [ia_GRID_phys], THD/1, RMS Measurement/1, Scope3/1
  Voltage Measurement1/1 -> [Vb_TNPC_phys], Scope1/2
  [S4a] -> IGBT/Diode5/1
  Voltage Measurement5/1 -> [VccT_TNPC_phys]
  [S4b] -> IGBT/Diode6/1
  [S1a] -> IGBT/Diode/1
  [S1c] -> IGBT/Diode4/1
  Current Measurement7/1 -> [ib_GRID_phys]
  [S4c] -> IGBT/Diode7/1
  Voltage Measurement2/1 -> [Va_TNPC_phys], Scope1/1
  Current Measurement8/1 -> [ic_GRID_phys]
  [S1b] -> IGBT/Diode3/1
  Current Measurement/1 -> Scope2/1, [ia_TNPC_phys]
  Voltage Measurement4/1 -> [VccB_TNPC_phys]
  CBPWM/1(Out1) -> [S1a]
  CBPWM/6(Out12) -> [S4c]
  [m_a] -> CBPWM/1(ma)
  [m_c] -> CBPWM/3(mc)
  CBPWM/3(Out6) -> [S1b]
  CBPWM/2(Out2) -> [S4a]
  CBPWM/4(Out7) -> [S4b]
  CBPWM/5(Out11) -> [S1c]
  [m_b] -> CBPWM/2(mb)
  Zero-Order Hold7/1 -> Data Type Conversion/1
  Zero-Order Hold1/1 -> Data Type Conversion1/1
  Zero-Order Hold2/1 -> Data Type Conversion2/1
  Zero-Order Hold3/1 -> Data Type Conversion3/1
  Zero-Order Hold4/1 -> Data Type Conversion4/1
  Zero-Order Hold5/1 -> Data Type Conversion5/1
  Zero-Order Hold6/1 -> Data Type Conversion6/1
  Zero-Order Hold8/1 -> Data Type Conversion7/1
  Zero-Order Hold9/1 -> Data Type Conversion8/1
  Zero-Order Hold10/1 -> Data Type Conversion9/1
  Zero-Order Hold11/1 -> Data Type Conversion10/1
  Data Type Conversion/1 -> Gain42/1
  Data Type Conversion1/1 -> Gain44/1
  Data Type Conversion2/1 -> Gain46/1
  Data Type Conversion3/1 -> Gain48/1
  Data Type Conversion4/1 -> Gain50/1
  Data Type Conversion5/1 -> Gain52/1
  Data Type Conversion6/1 -> Gain54/1
  Data Type Conversion7/1 -> Gain56/1
  Data Type Conversion8/1 -> Gain58/1
  Data Type Conversion9/1 -> Gain61/1
  Data Type Conversion10/1 -> Gain62/1
  Step/1 -> Enable_PQ_ctrl/Trigger
  Constant1/1 -> Enable_PQ_ctrl/1(In1)
  Step1/1 -> Enable_comp_ctrl/Trigger
  Constant3/1 -> Enable_comp_ctrl/1(In1)
  Step2/1 -> Enable_ctrl/Trigger
  Constant4/1 -> Enable_ctrl/1(In1)
  [p_osc_comp] -> PQref Calculation/5(p_osc_comp)
  [q_osc_comp] -> PQref Calculation/7(q_osc_comp)
  [q_avg_comp] -> PQref Calculation/6(q_avg_comp)
  Constant5/1 -> PQref Calculation/3(p_Vdc)
  Constant6/1 -> PQref Calculation/8(q_VoltVAr)
  [enable_comp] -> VoltVAr/3(enable)
  [vPCC_alpha] -> VoltVAr/1(v_alpha)
  [vPCC_beta] -> VoltVAr/2(v_beta)
  VoltVAr/1(V_rms) -> [V_rms]
  [V_rms] -> PQref Calculation/9(Voltage)
  [THD_i] -> PQref Calculation/10(THDi)
  VoltVAr/2(q_VoltVAr) -> Terminator/1
  Current Measurement3/1 -> [ic_load_phys]
  Current Measurement5/1 -> [ib_load_phys]
  Current Measurement4/1 -> [ia_load_phys]
  [ib_load_pu] -> MATLAB Function5/2(b)
  [ia_load_pu] -> MATLAB Function5/1(a)
  MATLAB Function5/2(beta) -> [il_beta]  "i_load_beta"
  MATLAB Function5/1(alpha) -> [il_alpha]  "i_load_alpha"
  [ic_load_pu] -> MATLAB Function5/3(c)
  [ia_TNPC_pu] -> Sum3/1
  [ia_GRID_pu] -> Sum3/2
  Sum3/1 -> Gain/1
  [ib_TNPC_pu] -> Sum4/1
  [ib_GRID_pu] -> Sum4/2
  Sum4/1 -> Gain1/1
  [ic_TNPC_pu] -> Sum5/1
  [ic_GRID_pu] -> Sum5/2
  Sum5/1 -> Gain2/1
  Gain/1 -> [ia_load_pu]
  Gain1/1 -> [ib_load_pu]
  Gain2/1 -> [ic_load_pu]
  Data Type Conversion12/1 -> Gain4/1
  Data Type Conversion11/1 -> Gain3/1
  From93/1 -> Zero-Order Hold12/1  "ia_GRID_phys"
  Zero-Order Hold12/1 -> Data Type Conversion11/1
  From92/1 -> Zero-Order Hold14/1  "ic_GRID_phys"
  Zero-Order Hold13/1 -> Data Type Conversion12/1
  Zero-Order Hold14/1 -> Data Type Conversion13/1
  From94/1 -> Zero-Order Hold13/1  "ib_GRID_phys"
  Data Type Conversion13/1 -> Gain5/1
  Gain3/1 -> Goto19/1
  Gain4/1 -> Goto24/1
  Gain5/1 -> Goto64/1
  RMS Measurement/1 -> Demux/1
  Demux/1 -> Scope11/1
  Demux/2 -> Scope5/1
  THD/1 -> Scope12/1
  [vPCC_alpha] -> MATLAB Function7/3(v_alpha)
  MATLAB Function8/4(q_osc) -> Scope13/4  "qO_EV"
  MATLAB Function7/2(p_osc) -> Scope16/2  "pO_GR"
  MATLAB Function6/1(p_avg) -> Scope15/1  "pA_L"
  MATLAB Function6/3(q_avg) -> Scope15/3  "qA_L"
  [iGRID_beta] -> MATLAB Function7/2(i_beta)
  MATLAB Function7/3(q_avg) -> [qa_GR], Scope16/3  "qA_GR"
  [vPCC_beta] -> MATLAB Function7/4(v_beta)
  [vPCC_alpha] -> MATLAB Function6/3(v_alpha)
  MATLAB Function6/2(p_osc) -> Scope15/2  "pO_L"
  MATLAB Function6/4(q_osc) -> Scope15/4  "qO_L"
  [vPCC_beta] -> MATLAB Function8/4(v_beta)
  MATLAB Function8/2(p_osc) -> Scope13/2  "pO_EV"
  MATLAB Function7/4(q_osc) -> Scope16/4  "qO_GR"
  [vPCC_beta] -> MATLAB Function6/4(v_beta)
  [iGRID_alpha] -> MATLAB Function7/1(i_alpha)
  [il_beta] -> MATLAB Function6/2(i_beta)
  MATLAB Function8/1(p_avg) -> Scope13/1  "pA_EV"
  [vPCC_alpha] -> MATLAB Function8/3(v_alpha)
  [iTNPC_alpha] -> MATLAB Function8/1(i_alpha)
  MATLAB Function8/3(q_avg) -> Scope13/3  "qA_EV"
  [il_alpha] -> MATLAB Function6/1(i_alpha)
  MATLAB Function7/1(p_avg) -> [pa_GR], Scope16/1  "pA_GR"
  [iTNPC_beta] -> MATLAB Function8/2(i_beta)
  MATLAB Function9/3(THDi) -> [THD_GR]
  MATLAB Function9/1(lambda_Q) -> [lQ_GR]
  [iGRID_alpha] -> MATLAB Function9/1(i_alpha)
  [iGRID_beta] -> MATLAB Function9/2(i_beta)
  [qa_GR] -> MATLAB Function9/6(q_avg)
  MATLAB Function9/2(lambda_PF) -> [lPF_GR]
  [vPCC_alpha] -> MATLAB Function9/3(v_alpha)
  [pa_GR] -> MATLAB Function9/5(p_avg)
  MATLAB Function9/4(S_fund) -> Scope14/1
  [vPCC_beta] -> MATLAB Function9/4(v_beta)
  [THD_GR] -> Gain6/1
  Gain6/1 -> Scope17/3  "THD"
  [lQ_GR] -> Scope17/1  "PF_Q"
  [lPF_GR] -> Scope17/2  "PF"
  [V_rms] -> Scope17/4  "V_rms"
  connections:
  Series RLC Branch1/LConn1 -- Voltage Measurement5/LConn1 -- IGBT/Diode3/LConn1 -- IGBT/Diode4/LConn1 -- IGBT/Diode/LConn1 -- DC Voltage Source/RConn1
  IGBT/Diode9/RConn1 -- Three-Phase Breaker1/LConn2 -- IGBT/Diode3/RConn1 -- IGBT/Diode6/LConn1
  Current Measurement5/LConn1 -- Series RLC Branch19/LConn1 -- Series RLC Branch15/LConn1 -- Series RLC Branch13/LConn1
  Series RLC Branch2/RConn1 -- Series RLC Branch5/LConn1 -- Series RLC Branch8/LConn1
  Series RLC Branch7/LConn1 -- Series RLC Branch10/LConn1 -- Series RLC Branch4/RConn1
  IGBT/Diode/RConn1 -- IGBT/Diode5/LConn1 -- IGBT/Diode1/RConn1 -- Three-Phase Breaker1/LConn1
  Voltage Measurement/LConn1 -- Current Measurement2/RConn1 -- Current Measurement3/RConn1 -- Current Measurement8/LConn1
  Voltage Measurement/LConn2 -- Ground2/LConn1 -- Voltage Measurement2/LConn2 -- Voltage Measurement1/LConn2
  Series RLC Branch9/RConn1 -- Series RLC Branch10/RConn1 -- Ground5/LConn1 -- Series RLC Branch8/RConn1
  Series RLC Branch3/RConn1 -- Series RLC Branch6/LConn1 -- Series RLC Branch9/LConn1
  IGBT/Diode4/RConn1 -- IGBT/Diode11/RConn1 -- IGBT/Diode7/LConn1 -- Three-Phase Breaker1/LConn3
  DC Voltage Source1/LConn1 -- IGBT/Diode5/RConn1 -- IGBT/Diode7/RConn1 -- IGBT/Diode6/RConn1 -- Voltage Measurement4/LConn2 -- Series RLC Branch11/RConn1
  IGBT/Diode2/RConn1 -- Voltage Measurement4/LConn1 -- Voltage Measurement5/LConn2 -- IGBT/Diode8/RConn1 -- IGBT/Diode10/RConn1 -- DC Voltage Source1/RConn1 -- DC Voltage Source/LConn1 -- Series RLC Branch11/LConn1 -- Series RLC Branch1/RConn1
  Series RLC Branch6/RConn1 -- Current Measurement1/LConn1
  Series RLC Branch2/LConn1 -- Three-Phase Breaker1/RConn1
  IGBT/Diode2/LConn1 -- IGBT/Diode1/LConn1
  Series RLC Branch7/RConn1 -- Current Measurement2/LConn1
  Current Measurement6/RConn1 -- AC Voltage Source2/RConn1
  AC Voltage Source1/RConn1 -- Current Measurement7/RConn1
  IGBT/Diode11/LConn1 -- IGBT/Diode10/LConn1
  Current Measurement/LConn1 -- Series RLC Branch5/RConn1
  Series RLC Branch3/LConn1 -- Three-Phase Breaker1/RConn2
  IGBT/Diode9/LConn1 -- IGBT/Diode8/LConn1
  Series RLC Branch4/LConn1 -- Three-Phase Breaker1/RConn3
  AC Voltage Source/RConn1 -- Current Measurement8/RConn1
  Series RLC Branch12/RConn1 -- Series RLC Branch14/RConn1 -- Series RLC Branch13/RConn1
  AC Voltage Source1/LConn1 -- AC Voltage Source2/LConn1 -- AC Voltage Source/LConn1 -- Ground1/LConn1
  Series RLC Branch17/RConn1 -- Series RLC Branch16/RConn1 -- Series RLC Branch15/RConn1
  Series RLC Branch/LConn1 -- Series RLC Branch18/LConn1 -- Universal Bridge/RConn1
  Series RLC Branch/RConn1 -- Universal Bridge/RConn2 -- Series RLC Branch18/RConn1
  Series RLC Branch20/RConn1 -- Universal Bridge/LConn3
  Series RLC Branch21/RConn1 -- Universal Bridge/LConn1
  Series RLC Branch19/RConn1 -- Universal Bridge/LConn2
  Current Measurement4/LConn1 -- Series RLC Branch12/LConn1 -- Series RLC Branch20/LConn1 -- Series RLC Branch16/LConn1
  Current Measurement7/LConn1 -- Voltage Measurement1/LConn1 -- Current Measurement5/RConn1 -- Current Measurement1/RConn1
  Current Measurement4/RConn1 -- Voltage Measurement2/LConn1 -- Current Measurement6/LConn1 -- Current Measurement/RConn1
  Series RLC Branch21/LConn1 -- Series RLC Branch17/LConn1 -- Series RLC Branch14/LConn1 -- Current Measurement3/LConn1

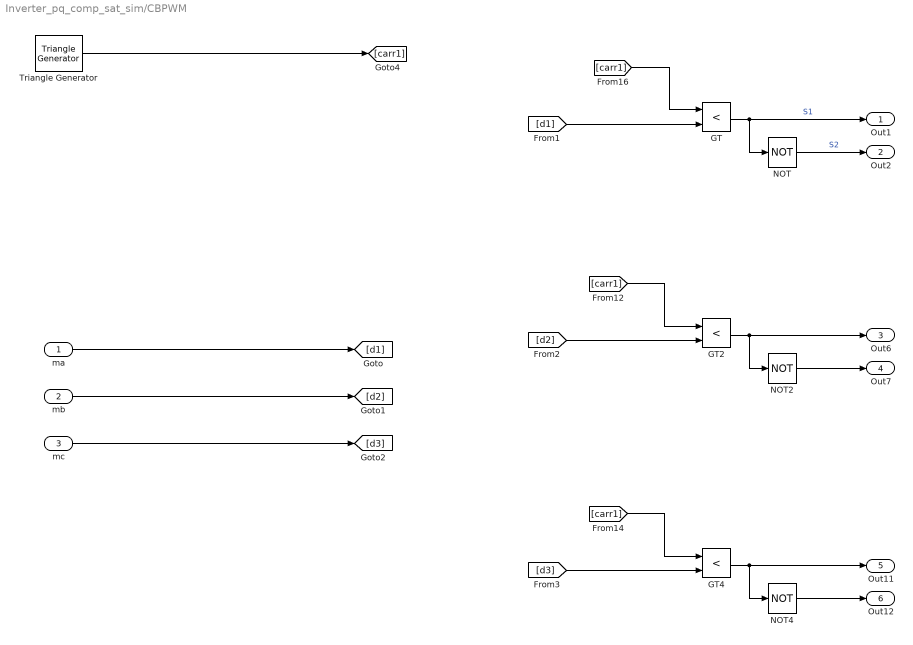
== system Inverter_pq_comp_sat_sim/CBPWM ==
  ma : Inport
  mb : Inport  Port=2
  mc : Inport  Port=3
  GT : RelationalOperator  Operator=<  OutDataTypeStr=boolean  RndMeth=Simplest  InputSameDT=off
  GT2 : RelationalOperator  Operator=<  OutDataTypeStr=boolean  RndMeth=Simplest  InputSameDT=off
  GT4 : RelationalOperator  Operator=<  OutDataTypeStr=boolean  RndMeth=Simplest  InputSameDT=off
  NOT : Logic  Operator=NOT  IconShape=distinctive  AllPortsSameDT=off  OutDataTypeStr=boolean
  NOT2 : Logic  Operator=NOT  IconShape=distinctive  AllPortsSameDT=off  OutDataTypeStr=boolean
  NOT4 : Logic  Operator=NOT  IconShape=distinctive  AllPortsSameDT=off  OutDataTypeStr=boolean
  Triangle Generator : spsTriangleGeneratorLib/Triangle Generator  Freq=fs  Phase=0  Ts=Tstep
  Out1 : Outport
  Out2 : Outport  Port=2
  Out6 : Outport  Port=3
  Out7 : Outport  Port=4
  Out11 : Outport  Port=5
  Out12 : Outport  Port=6
  wires:
  NOT2/1 -> Out7/1
  [carr1] -> GT4/1
  GT4/1 -> Out11/1, NOT4/1
  [carr1] -> GT2/1
  GT/1 -> Out1/1, NOT/1  "S1"
  [carr1] -> GT/1
  GT2/1 -> Out6/1, NOT2/1
  NOT/1 -> Out2/1  "S2"
  NOT4/1 -> Out12/1
  ma/1 -> [d1]
  mb/1 -> [d2]
  [d1] -> GT/2
  [d2] -> GT2/2
  [d3] -> GT4/2
  Triangle Generator/1 -> [carr1]
  mc/1 -> [d3]

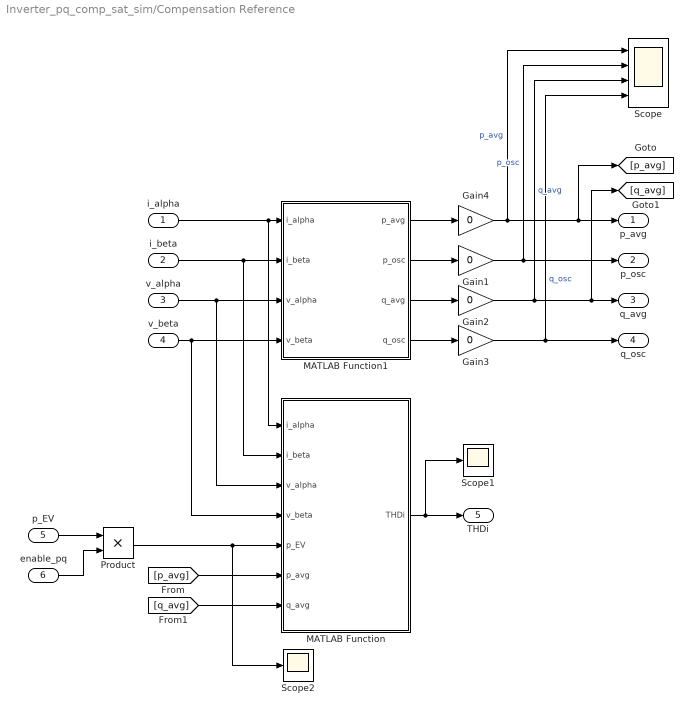
== system Inverter_pq_comp_sat_sim/Compensation Reference ==
  i_alpha : Inport
  i_beta : Inport  Port=2
  v_alpha : Inport  Port=3
  v_beta : Inport  Port=4
  p_EV : Inport  Port=5
  enable_pq : Inport  Port=6
  Gain{1..4} (4 alike) : Gain  Gain=0
  MATLAB Function : MATLAB Function  TreatAsAtomicUnit=on
  MATLAB Function1 : MATLAB Function  TreatAsAtomicUnit=on
  Product : Product
  Scope : Scope  NumInputPorts=4
  Scope1 : Scope
  Scope2 : Scope
  p_avg : Outport
  p_osc : Outport  Port=2
  q_avg : Outport  Port=3
  q_osc : Outport  Port=4
  THDi : Outport  Port=5
  wires:
  MATLAB Function1/1(p_avg) -> Gain4/1
  MATLAB Function1/3(q_avg) -> Gain2/1
  MATLAB Function1/2(p_osc) -> Gain1/1
  i_alpha/1 -> MATLAB Function/1(i_alpha), MATLAB Function1/1(i_alpha)
  MATLAB Function1/4(q_osc) -> Gain3/1
  i_beta/1 -> MATLAB Function/2(i_beta), MATLAB Function1/2(i_beta)
  v_alpha/1 -> MATLAB Function/3(v_alpha), MATLAB Function1/3(v_alpha)
  v_beta/1 -> MATLAB Function/4(v_beta), MATLAB Function1/4(v_beta)
  Gain4/1 -> Scope/1, [p_avg], p_avg/1  "p_avg"
  Gain1/1 -> Scope/2, p_osc/1  "p_osc"
  Gain2/1 -> Scope/3, [q_avg], q_avg/1  "q_avg"
  Gain3/1 -> Scope/4, q_osc/1  "q_osc"
  [p_avg] -> MATLAB Function/6(p_avg)
  [q_avg] -> MATLAB Function/7(q_avg)
  MATLAB Function/1(THDi) -> Scope1/1, THDi/1
  Product/1 -> Scope2/1, MATLAB Function/5(p_EV)
  p_EV/1 -> Product/1
  enable_pq/1 -> Product/2

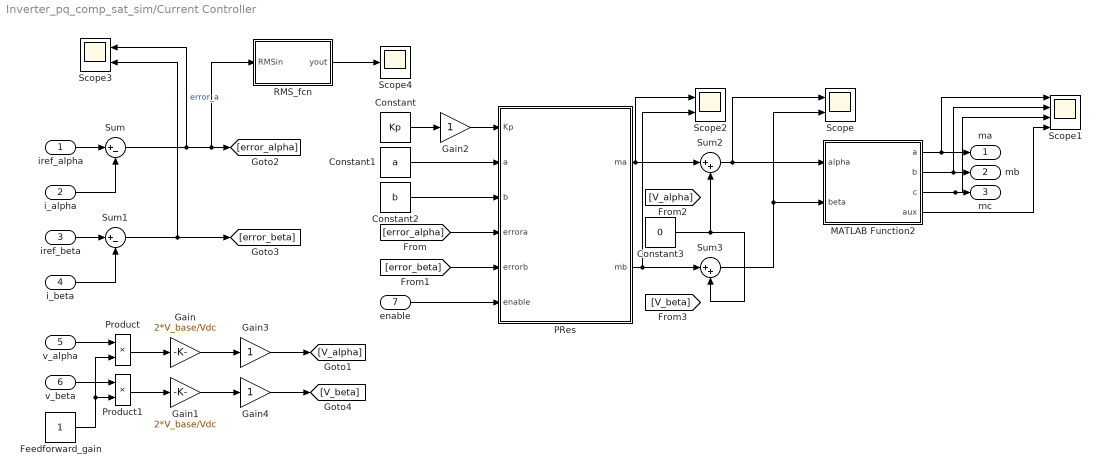
== system Inverter_pq_comp_sat_sim/Current Controller ==
  iref_alpha : Inport
  i_alpha : Inport  Port=2
  iref_beta : Inport  Port=3
  i_beta : Inport  Port=4
  v_alpha : Inport  Port=5
  v_beta : Inport  Port=6
  enable : Inport  Port=7
  Constant : Constant  Value=Kp  OutDataTypeStr=single
  Constant1 : Constant  Value=a  OutDataTypeStr=single
  Constant2 : Constant  Value=b  OutDataTypeStr=single
  Constant3 : Constant  Value=0  OutDataTypeStr=single
  Feedforward_gain : Constant  OutDataTypeStr=single
  Gain : Gain  Gain=2*V_base/Vdc
  Gain1 : Gain  Gain=2*V_base/Vdc
  Gain2 : Gain
  Gain3 : Gain
  Gain4 : Gain
  MATLAB Function2 : MATLAB Function  TreatAsAtomicUnit=on
  PRes : MATLAB Function  TreatAsAtomicUnit=on
  Product : Product
  Product1 : Product
  RMS_fcn : MATLAB Function  TreatAsAtomicUnit=on
  Scope : Scope  NumInputPorts=2
  Scope1 : Scope  NumInputPorts=4
  Scope2 : Scope  NumInputPorts=2
  Scope3 : Scope  NumInputPorts=2
  Scope4 : Scope
  Sum : Sum  Inputs=|+-
  Sum1 : Sum  Inputs=|+-
  Sum2 : Sum  Inputs=|++
  Sum3 : Sum  Inputs=|++
  ma : Outport
  mb : Outport  Port=2
  mc : Outport  Port=3
  wires:
  Constant1/1 -> PRes/2(a)
  Constant2/1 -> PRes/3(b)
  [error_alpha] -> PRes/4(errora)
  [error_beta] -> PRes/5(errorb)
  iref_alpha/1 -> Sum/1
  i_alpha/1 -> Sum/2
  iref_beta/1 -> Sum1/1
  i_beta/1 -> Sum1/2
  Sum1/1 -> [error_beta], Scope3/2
  Sum/1 -> Scope3/1, RMS_fcn/1(RMSin), [error_alpha]  "error_a"
  enable/1 -> PRes/6(enable)
  PRes/1(ma) -> Scope2/1, Sum2/1
  Sum2/1 -> Scope/1, MATLAB Function2/1(alpha)
  PRes/2(mb) -> Scope2/2, Sum3/1
  v_beta/1 -> Product1/1
  Product1/1 -> Gain1/1
  v_alpha/1 -> Product/1
  Product/1 -> Gain/1
  Feedforward_gain/1 -> Product/2, Product1/2
  Constant/1 -> Gain2/1
  MATLAB Function2/1(a) -> Scope1/1, ma/1
  MATLAB Function2/2(b) -> Scope1/2, mb/1
  MATLAB Function2/3(c) -> Scope1/3, mc/1
  MATLAB Function2/4(aux) -> Scope1/4
  Sum3/1 -> Scope/2, MATLAB Function2/2(beta)
  Gain/1 -> Gain3/1
  Gain1/1 -> Gain4/1
  Gain2/1 -> PRes/1(Kp)
  Gain3/1 -> [V_alpha]
  Gain4/1 -> [V_beta]
  RMS_fcn/1(yout) -> Scope4/1
  Constant3/1 -> Sum3/2, Sum2/2

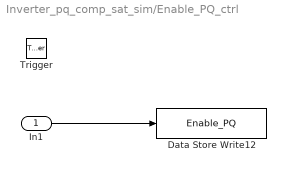
== system Inverter_pq_comp_sat_sim/Enable_PQ_ctrl ==
  In1 : Inport
  Trigger : TriggerPort  VariantControl=(inherit)
  Data Store Write12 : DataStoreWrite  DataStoreName=Enable_PQ  IndexOptions=Index vector (dialog)  Indices=1  OutputSizes=1
  wires:
  In1/1 -> Data Store Write12/1

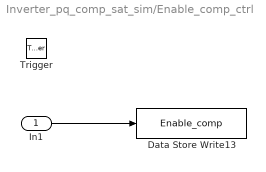
== system Inverter_pq_comp_sat_sim/Enable_comp_ctrl ==
  In1 : Inport
  Trigger : TriggerPort  VariantControl=(inherit)
  Data Store Write13 : DataStoreWrite  DataStoreName=Enable_comp  IndexOptions=Index vector (dialog)  Indices=1  OutputSizes=1
  wires:
  In1/1 -> Data Store Write13/1

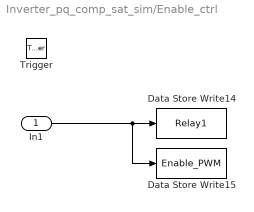
== system Inverter_pq_comp_sat_sim/Enable_ctrl ==
  In1 : Inport
  Trigger : TriggerPort  VariantControl=(inherit)
  Data Store Write14 : DataStoreWrite  DataStoreName=Relay1  IndexOptions=Index vector (dialog)  Indices=1  OutputSizes=1
  Data Store Write15 : DataStoreWrite  DataStoreName=Enable_PWM  IndexOptions=Index vector (dialog)  Indices=1  OutputSizes=1
  wires:
  In1/1 -> Data Store Write15/1, Data Store Write14/1
